simulink model "REAL_THREE_TANK"  (R2025b)
settings: Solver=ode15s  StartTime=0.0  StopTime=1500  RelTol=1e-3
InitFcn:
  | run("index.m")
StopFcn:
  | data_name = "realtime_data";
  | save_name = format_file_name(data_name,true);
  | 
  | % Save output data
  | save(save_name,"out")
values from neighbouring files (symbols this model uses):
  adaptParam = 0.15    [index.m]
  hiddenStates = 0    [index.m]
  model_const = struct()    [index.m]
undefined symbols (not defined in the file or in its folder): CR, LF, sigbuilder_block
libraries: instrumentseriallib x3, simulink x1
(part 1 of 2)
settings Model: Creator=HP  LastModifiedBy=USER PC
settings RTWCC: GPUComputeCapability=3.5
settings GRTTargetCC: ArrayLayout=Row-major

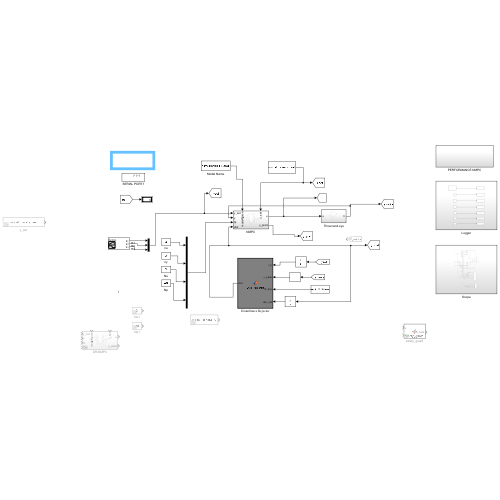
[thumbnail: Simulink's stored preview of the top-level diagram]
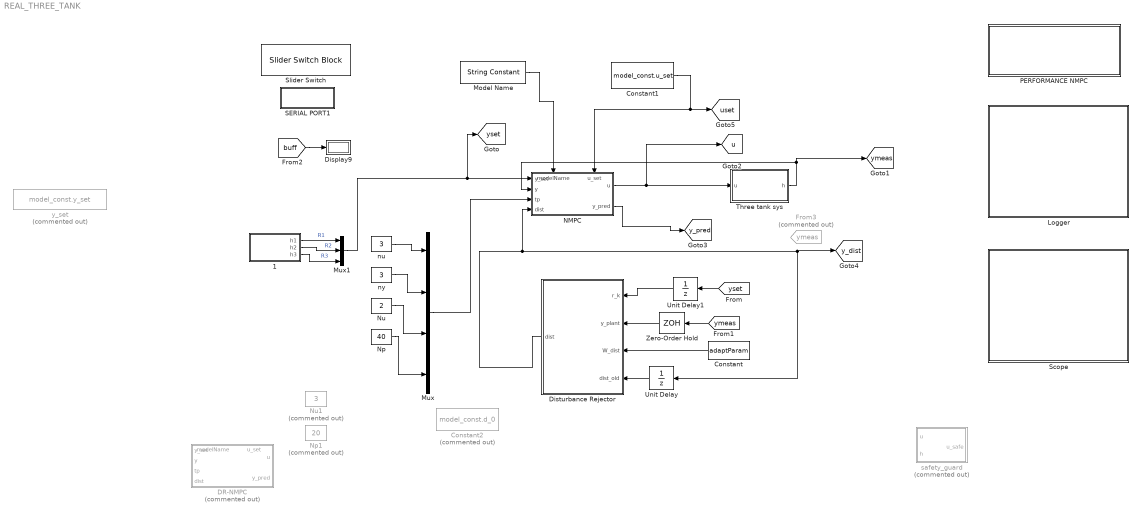
== system REAL_THREE_TANK ==
  " 1" : Subsystem  Tag=STV Subsys  LoadFcn=sigbuilder_block('load');  StartFcn=sigbuilder_block('start');  StopFcn=sigbuilder_block('stop');  ClipboardFcn=sigbuilder_block('clipboard');  mask(Sigbuilder block){tuvar=[0:10]}
      mask help: Simulink:masks:SigbuilderBlock_MD
      mask init:
      | if ~strcmp(get_param(bdroot(gcbh),'SimulationStatus'),'stopped') tuvar = sigbuilder_block('maskInit'); end
      settings: CopyFcn=sigbuilder_block('copy');  DeleteFcn=sigbuilder_block('delete');  ModelCloseFcn=sigbuilder_block('modelClose');  PreSaveFcn=sigbuilder_block('preSave');  PauseFcn=sigbuilder_block('pause');  ContinueFcn=sigbuilder_block('continue');  NameChangeFcn=sigbuilder_block('namechange');  OpenFcn=sigbuilder_block('open',[316.5 171.75 805.5 485.25 ]);  CloseFcn=sigbuilder_block('close');
      mask Display: plot(0, 0, 100, 100,[2, 2, 32, 32, 2], [68, 8, 8, 68, 68],[32, 2], [38, 38], [32, 19, 2],[53, 60, 44], [32, 17, 17, 2],[16, 16, 31, 31]);txt = getActiveGroup(gcbh);text(2, 100, txt,'verticalAlignment', 'top');
  Constant : Constant  Value=adaptParam
  Constant1 : Constant  Value=model_const.u_set  SampleTime=model_const.ts
  Constant2 : Constant  Commented=on  Value=model_const.d_0  SampleTime=model_const.ts
  DR-NMPC : Subsystem  Commented=on
      settings: PortSchema="{\"entries\":[{\"content\":{\"sides\":[{\"content\":{\"connectorIds\":[\"In1\",\"In2\",\"In3\",\"In4\"]},\"type\":\"ConnectorPlacement.EquallySpacedRectSide\",\"uuid\":\"b907109f-bf70-45ef-b014-879f3ccfb12e\"},{\"content\":{\"connectorIds\":[\"Out1\",\"Out2\"],\"side\":\"RIGHT\"},\"type\":\"ConnectorPlacement.EquallySpacedRectSide\",\"uuid\":\"26d01547-fbc3-4b4e-b6e6-c22ae9e5b6d6\"},{\"content\":{\"connectorIds\":[\"In5\",\"In6\"],\"side\":\"TOP\"},\"type\":\"ConnectorPlacement.EquallySpacedRectSide\",\"uuid\":\"f1d5a2c8-1fb2-4706-a136-ec661fe312a9\"}]},\"type\":\"ConnectorPlacement.EquallySpacedConnector\",\"uuid\":\"8e79e654-12d3-4871-a9fc-130c68b7f74a\"}],\"packageUris\":[\"http://schema.mathworks.com/mf0/Connector/R2020b\"],\"version\":\"1.0\"}"
  Display9 : Display
  Disturbance Rejector : MATLAB Function  TreatAsAtomicUnit=on  SystemSampleTime=10
  From3 : From  Commented=on  GotoTag=ymeas  TagVisibility=global
  Logger : Subsystem
  Model Name : StringConstant  String=networkModelName
  Mux : Mux
  Mux1 : Mux  Inputs=3
  NMPC : Subsystem
      settings: PortSchema="{\"entries\":[{\"content\":{\"sides\":[{\"content\":{\"connectorIds\":[\"In1\",\"In2\",\"In3\",\"In4\"]},\"type\":\"ConnectorPlacement.EquallySpacedRectSide\",\"uuid\":\"b907109f-bf70-45ef-b014-879f3ccfb12e\"},{\"content\":{\"connectorIds\":[\"Out1\",\"Out2\"],\"side\":\"RIGHT\"},\"type\":\"ConnectorPlacement.EquallySpacedRectSide\",\"uuid\":\"26d01547-fbc3-4b4e-b6e6-c22ae9e5b6d6\"},{\"content\":{\"connectorIds\":[\"In5\",\"In6\"],\"side\":\"TOP\"},\"type\":\"ConnectorPlacement.EquallySpacedRectSide\",\"uuid\":\"f1d5a2c8-1fb2-4706-a136-ec661fe312a9\"}]},\"type\":\"ConnectorPlacement.EquallySpacedConnector\",\"uuid\":\"8e79e654-12d3-4871-a9fc-130c68b7f74a\"}],\"packageUris\":[\"http://schema.mathworks.com/mf0/Connector/R2020b\"],\"version\":\"1.0\"}"
  Np : Constant  Value=40
  Np1 : Constant  Commented=on  Value=20
  Nu : Constant  Value=2
  Nu1 : Constant  Commented=on  Value=3
  PERFORMANCE NMPC : Subsystem
  SERIAL PORT1 : Subsystem
      mask Display: image('rs232.png');
  Scope : Subsystem
  Slider Switch : SliderSwitchBlock  LabelPosition=Hide
  Three tank sys : Subsystem
  Unit Delay : UnitDelay  InitialCondition=[0;0;0]  SampleTime=model_const.ts  HasFrameUpgradeWarning=on
  Unit Delay1 : UnitDelay  InitialCondition=[100; 0.4; 0.2]  SampleTime=model_const.ts  HasFrameUpgradeWarning=on
  Zero-Order Hold : ZeroOrderHold  SampleTime=model_const.ts
  nu : Constant  Value=3
  ny : Constant  Value=3
  safety_guard : MATLAB Function  Commented=on  TreatAsAtomicUnit=on
  y_set : Constant  Commented=on  Value=model_const.y_set  SampleTime=model_const.ts  LockScale=on
  tag scope: u=global, uset=global, y_dist=global, y_pred=global, ymeas=global, yset=global
  wires:
  Nu/1 -> Mux/3
  Constant/1 -> Disturbance Rejector/3(W_dist)
  Unit Delay/1 -> Disturbance Rejector/4(dist_old)
  Mux/1 -> NMPC/3(tp)
  Np/1 -> Mux/4
  [ymeas] -> Zero-Order Hold/1
  Model Name/1 -> NMPC/5(modelName)
  nu/1 -> Mux/1
  ny/1 -> Mux/2
  Constant1/1 -> NMPC/6(u_set), [uset]
  Disturbance Rejector/1(dist) -> NMPC/4(dist), [y_dist], Unit Delay/1
  [yset] -> Unit Delay1/1
  Three tank sys/1(h) -> NMPC/2(y), [ymeas]
  [buff] -> Display9/1
  " 1"/3(h3) -> Mux1/3  "R3"
  " 1"/2(h2) -> Mux1/2  "R2"
  " 1"/1(h1) -> Mux1/1  "R1"
  NMPC/2(y_pred) -> [y_pred]
  NMPC/1(u) -> Three tank sys/1(u), [u]
  Mux1/1 -> [yset], NMPC/1(y_set)
  Zero-Order Hold/1 -> Disturbance Rejector/2(y_plant)
  Unit Delay1/1 -> Disturbance Rejector/1(r_k)

== system REAL_THREE_TANK/ 1 ==
  Demux : Demux  Tag=STV Demux  Outputs=3
      settings: DisplayOption=none
  FromWs : FromWorkspace  Tag=STV FromWs  VariableName=tuvar  SampleTime=1
      SigBuilderData=|
      | common.afterFinalStr = 'Extrapolate'
      | common.sampleTime = '1'
      | dataSet.timeRange = [0 1500]
      | dataSet.name = 'Servo'
      | sbobj.Groups.Name = 'Servo'
      | sbobj.Groups.Signals(1).Name = 'h1'
      | sbobj.Groups.Signals(1).XData = [0 400 400 1500]
      | sbobj.Groups.Signals(1).YData = [14.29 14.29 20 20]
      | sbobj.Groups.Signals(2).Name = 'h2'
      | sbobj.Groups.Signals(2).XData = [0 800 800 1500]
      | sbobj.Groups.Signals(2).YData = [13.51 13.51 20 20]
      | sbobj.Groups.Signals(3).Name = 'h3'
      | sbobj.Groups.Signals(3).XData = [0 1200 1200 1500]
      | sbobj.Groups.Signals(3).YData = [16.06 16.06 20 20]
      | sbobj.Groups.TimeRange = [0 1500]
  h1 : Outport  Tag=STV Outport  VectorParamsAs1DForOutWhenUnconnected=off
  h2 : Outport  Tag=STV Outport  Port=2  VectorParamsAs1DForOutWhenUnconnected=off
  h3 : Outport  Tag=STV Outport  Port=3  VectorParamsAs1DForOutWhenUnconnected=off
  wires:
  FromWs/1 -> Demux/1
  Demux/1 -> h1/1
  Demux/2 -> h2/1
  Demux/3 -> h3/1

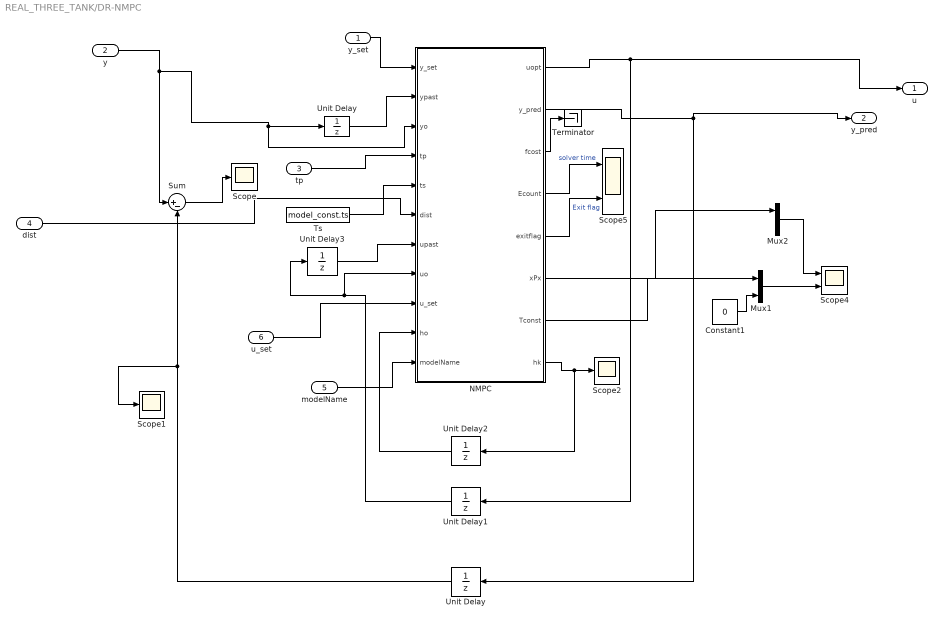
== system REAL_THREE_TANK/DR-NMPC ==
  y_set : Inport
  y : Inport  Port=2
  tp : Inport  Port=3
  dist : Inport  Port=4
  modelName : Inport  Port=5
  u_set : Inport  Port=6
  "  Unit Delay  " : UnitDelay  InitialCondition=model_const.y_0  SampleTime=model_const.ts  HasFrameUpgradeWarning=on
  " Unit Delay " : UnitDelay  InitialCondition=model_const.y_set  SampleTime=model_const.ts  HasFrameUpgradeWarning=on
  Constant1 : Constant  Value=0
  Mux1 : Mux  Inputs=2
  Mux2 : Mux  Inputs=2
  "NMPC " : MATLAB Function  TreatAsAtomicUnit=on  SystemSampleTime=model_const.ts
  Scope : Scope
      settings: ActiveDisplayYMinimum=-0.81983  ActiveDisplayYMaximum=1.85991
  Scope1 : Scope
      settings: ActiveDisplayYMinimum=2.45433  ActiveDisplayYMaximum=11.20291
  Scope2 : Scope
      settings: ActiveDisplayYMinimum=-0.0970614142715931  ActiveDisplayYMaximum=0.12913854792714119
  Scope4 : Scope  NumInputPorts=2
      settings: ActiveDisplayYMinimum=-0.25  ActiveDisplayYMaximum=2.25  DataLoggingVariableName=ScopeData2
  Scope5 : Scope  NumInputPorts=2
      settings: ShowGrid=off  ActiveDisplayYMinimum=-2.5  ActiveDisplayYMaximum=2.5  DataLoggingVariableName=ScopeData3
  Sum : Sum  Inputs=|+-
  "Terminator " : Terminator
  Ts : Constant  Value=model_const.ts
  Unit Delay1 : UnitDelay  InitialCondition=model_const.u_0  SampleTime=model_const.ts  HasFrameUpgradeWarning=on
  Unit Delay2 : UnitDelay  InitialCondition=hiddenStates  SampleTime=model_const.ts  HasFrameUpgradeWarning=on
  Unit Delay3 : UnitDelay  InitialCondition=model_const.u_0  SampleTime=model_const.ts  HasFrameUpgradeWarning=on
  u : Outport  VectorParamsAs1DForOutWhenUnconnected=off
  y_pred : Outport  Port=2  VectorParamsAs1DForOutWhenUnconnected=off
  wires:
  y_set/1 -> "NMPC "/1(y_set)
  tp/1 -> "NMPC "/4(tp)
  Ts/1 -> "NMPC "/5(ts)
  "NMPC "/3(fcost) -> "Terminator "/1
  y/1 -> Sum/1, "NMPC "/3(yo), " Unit Delay "/1
  "  Unit Delay  "/1 -> Scope1/1, Sum/2
  Sum/1 -> Scope/1
  dist/1 -> "NMPC "/6(dist)
  Constant1/1 -> Mux1/2
  Mux2/1 -> Scope4/1
  Mux1/1 -> Scope4/2
  "NMPC "/7(Tconst) -> Mux1/1
  "NMPC "/6(xPx) -> Mux2/1
  "NMPC "/4(Ecount) -> Scope5/1  "solver time"
  "NMPC "/5(exitflag) -> Scope5/2  "Exit flag"
  "NMPC "/8(hk) -> Unit Delay2/1, Scope2/1
  Unit Delay2/1 -> "NMPC "/10(ho)
  modelName/1 -> "NMPC "/11(modelName)
  "NMPC "/1(uopt) -> Unit Delay1/1, u/1
  Unit Delay1/1 -> Unit Delay3/1, "NMPC "/8(uo)
  " Unit Delay "/1 -> "NMPC "/2(ypast)
  Unit Delay3/1 -> "NMPC "/7(upast)
  u_set/1 -> "NMPC "/9(u_set)
  "NMPC "/2(y_pred) -> y_pred/1, "  Unit Delay  "/1

== system REAL_THREE_TANK/Logger ==
  String Constant : StringConstant  String=description
  To Workspace : ToWorkspace  VariableName=input  SaveFormat=Structure With Time  SampleTime=3
      settings: Decimation=2
  To Workspace1 : ToWorkspace  VariableName=desc  SaveFormat=Structure With Time  SampleTime=3
      settings: Decimation=2
  To Workspace2 : ToWorkspace  VariableName=input_set  SaveFormat=Structure With Time  SampleTime=3
      settings: Decimation=2
  To Workspace3 : ToWorkspace  VariableName=out_dist  SaveFormat=Structure With Time  SampleTime=3
      settings: Decimation=2
  To Workspace4 : ToWorkspace  VariableName=out_pred  SaveFormat=Structure With Time  SampleTime=3
      settings: Decimation=2
  To Workspace5 : ToWorkspace  VariableName=out_meas  SaveFormat=Structure With Time  SampleTime=3
      settings: Decimation=2
  To Workspace6 : ToWorkspace  VariableName=out_set  SaveFormat=Structure With Time  SampleTime=3
      settings: Decimation=2
  wires:
  [u] -> To Workspace/1
  [yset] -> To Workspace6/1
  [ymeas] -> To Workspace5/1
  [y_pred] -> To Workspace4/1
  [y_dist] -> To Workspace3/1
  [uset] -> To Workspace2/1
  String Constant/1 -> To Workspace1/1

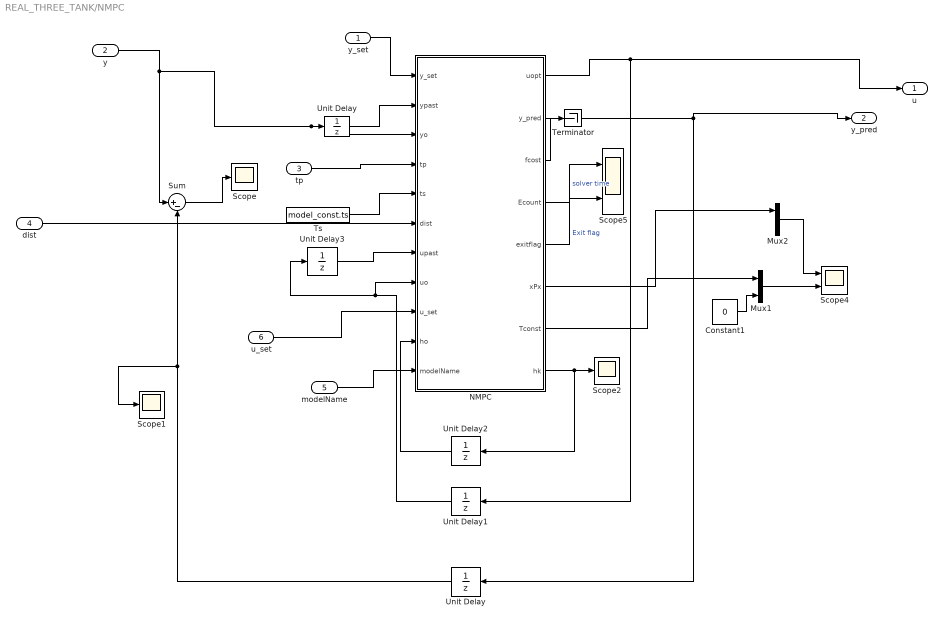
== system REAL_THREE_TANK/NMPC ==
  y_set : Inport
  y : Inport  Port=2
  tp : Inport  Port=3
  dist : Inport  Port=4
  modelName : Inport  Port=5
  u_set : Inport  Port=6
  "  Unit Delay  " : UnitDelay  InitialCondition=model_const.y_0  SampleTime=model_const.ts  HasFrameUpgradeWarning=on
  " Unit Delay " : UnitDelay  InitialCondition=[0 0 0]  SampleTime=model_const.ts  HasFrameUpgradeWarning=on
  Constant1 : Constant  Value=0
  Mux1 : Mux  Inputs=2
  Mux2 : Mux  Inputs=2
  "NMPC " : MATLAB Function  TreatAsAtomicUnit=on  SystemSampleTime=model_const.ts
  Scope : Scope
      settings: ActiveDisplayYMinimum=-0.81983  ActiveDisplayYMaximum=1.85991
  Scope1 : Scope
      settings: ActiveDisplayYMinimum=2.45433  ActiveDisplayYMaximum=11.20291
  Scope2 : Scope
      settings: ActiveDisplayYMinimum=-0.0970614142715931  ActiveDisplayYMaximum=0.12913854792714119
  Scope4 : Scope  NumInputPorts=2
      settings: ActiveDisplayYMinimum=-0.25  ActiveDisplayYMaximum=2.25  DataLoggingVariableName=ScopeData2
  Scope5 : Scope  NumInputPorts=2
      settings: ShowGrid=off  ActiveDisplayYMinimum=-2.5  ActiveDisplayYMaximum=2.5  DataLoggingVariableName=ScopeData3
  Sum : Sum  Inputs=|+-
  "Terminator " : Terminator
  Ts : Constant  Value=model_const.ts
  Unit Delay1 : UnitDelay  InitialCondition=model_const.u_0  SampleTime=model_const.ts  HasFrameUpgradeWarning=on
  Unit Delay2 : UnitDelay  InitialCondition=hiddenStates  SampleTime=model_const.ts  HasFrameUpgradeWarning=on
  Unit Delay3 : UnitDelay  InitialCondition=model_const.u_0  SampleTime=model_const.ts  HasFrameUpgradeWarning=on
  u : Outport  VectorParamsAs1DForOutWhenUnconnected=off
  y_pred : Outport  Port=2  VectorParamsAs1DForOutWhenUnconnected=off
  wires:
  y_set/1 -> "NMPC "/1(y_set)
  tp/1 -> "NMPC "/4(tp)
  Ts/1 -> "NMPC "/5(ts)
  "NMPC "/3(fcost) -> "Terminator "/1
  y/1 -> Sum/1, "NMPC "/3(yo), " Unit Delay "/1
  "  Unit Delay  "/1 -> Scope1/1, Sum/2
  Sum/1 -> Scope/1
  dist/1 -> "NMPC "/6(dist)
  Constant1/1 -> Mux1/2
  Mux2/1 -> Scope4/1
  Mux1/1 -> Scope4/2
  "NMPC "/7(Tconst) -> Mux1/1
  "NMPC "/6(xPx) -> Mux2/1
  "NMPC "/4(Ecount) -> Scope5/1  "solver time"
  "NMPC "/5(exitflag) -> Scope5/2  "Exit flag"
  "NMPC "/8(hk) -> Unit Delay2/1, Scope2/1
  Unit Delay2/1 -> "NMPC "/10(ho)
  modelName/1 -> "NMPC "/11(modelName)
  "NMPC "/1(uopt) -> Unit Delay1/1, u/1
  Unit Delay1/1 -> Unit Delay3/1, "NMPC "/8(uo)
  " Unit Delay "/1 -> "NMPC "/2(ypast)
  Unit Delay3/1 -> "NMPC "/7(upast)
  u_set/1 -> "NMPC "/9(u_set)
  "NMPC "/2(y_pred) -> y_pred/1, "  Unit Delay  "/1

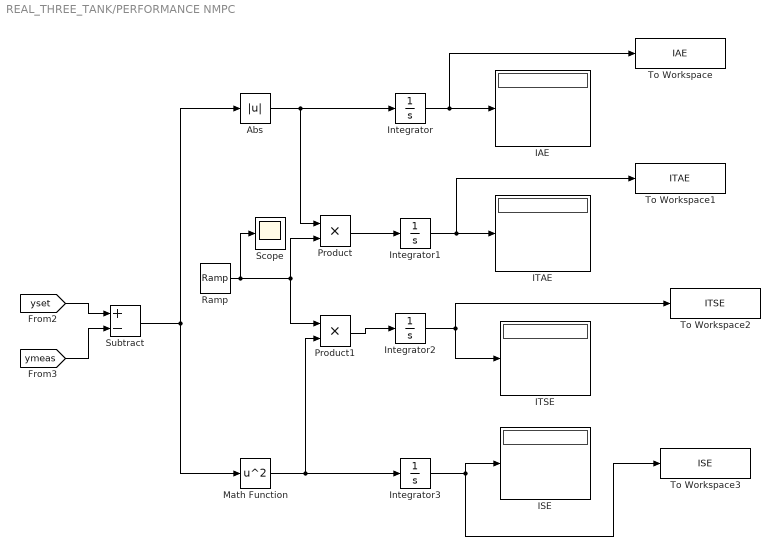
== system REAL_THREE_TANK/PERFORMANCE NMPC ==
  Abs : Abs  SaturateOnIntegerOverflow=off
  IAE : Display
  ISE : Display
  ITAE : Display
  ITSE : Display
  Integrator{,1..3} (4 alike) : Integrator
  Math Function : Math  Operator=square  SignedPower=on
  Product : Product  RndMeth=Zero
  Product1 : Product  RndMeth=Zero
  Ramp : simulink/Sources/Ramp  slope=1  start=0  InitialOutput=0
  Scope : Scope
      settings: DataLoggingSaveFormat=Array
  Subtract : Sum  Inputs=+-
  To Workspace : ToWorkspace  VariableName=IAE  SaveFormat=Structure With Time  SampleTime=3
      settings: Decimation=4
  To Workspace1 : ToWorkspace  VariableName=ITAE  SaveFormat=Structure With Time  SampleTime=3
      settings: Decimation=4
  To Workspace2 : ToWorkspace  VariableName=ITSE  SaveFormat=Structure With Time  SampleTime=3
      settings: Decimation=4
  To Workspace3 : ToWorkspace  VariableName=ISE  SaveFormat=Structure With Time  SampleTime=3
      settings: Decimation=4
  wires:
  Integrator1/1 -> To Workspace1/1, ITAE/1
  Integrator3/1 -> ISE/1, To Workspace3/1
  Product/1 -> Integrator1/1
  Product1/1 -> Integrator2/1
  Math Function/1 -> Product1/2, Integrator3/1
  Ramp/1 -> Scope/1, Product1/1, Product/2
  Integrator/1 -> To Workspace/1, IAE/1
  Abs/1 -> Product/1, Integrator/1
  Subtract/1 -> Abs/1, Math Function/1
  [yset] -> Subtract/1
  [ymeas] -> Subtract/2
  Integrator2/1 -> ITSE/1, To Workspace2/1

== system REAL_THREE_TANK/SERIAL PORT1 ==
  Display : Display
  Serial Configuration : instrumentseriallib/Serial Configuration  Priority=-200000  PortSel=COM10  Port=COM10  ComPort=COM10  BaudRate=115200  DataBits=8  Parity=none  StopBits=1  ByteOrder=little-endian  FlowControl=none  Timeout=3000  SimulateUsing=Interpreted execution  BlockInModel=on  aMode=1
  Serial Receive : instrumentseriallib/Serial Receive  Priority=1  PortSel=COM10  Port=COM10  ComPort=COM10  DataType=int8  SaveDataType=uint8  ToggleHeader=on  Header=[35 35]  ToggleDataSize=on  DataSize=[1 15]  ToggleTerminator=on  Terminator=CR/LF ('\r\n')  CustomTerminator=[]  InputFormat=Column major  EnableBlockingMode=off  ActionDataUnavailable=Output last received value  ActionWhenDataUnavailable=Output last received value  CustomValue=0  SampleTime=1  SimulateUsing=Interpreted execution  BlockInModel=on  aMode=1  LibraryInUse=instrumentlib
  Serial Send : instrumentseriallib/Serial Send  Priority=1  PortSel=COM10  Port=COM10  ComPort=COM10  Header=[]  Terminator=<none>  CustomTerminator=[]  EnableBlockingMode=on  SimulateUsing=Interpreted execution  BlockInModel=on  aMode=1
  To Workspace : ToWorkspace  VariableName=raw_read_sensor  SaveFormat=Structure With Time  SampleTime=-1
  To Workspace1 : ToWorkspace  VariableName=raw_read_status  SaveFormat=Structure With Time  SampleTime=-1
  tag scope: buff=global, rcv=global
  wires:
  Serial Receive/1 -> [rcv], To Workspace/1
  [send] -> Serial Send/1
  Serial Receive/2 -> To Workspace1/1, [buff], Display/1

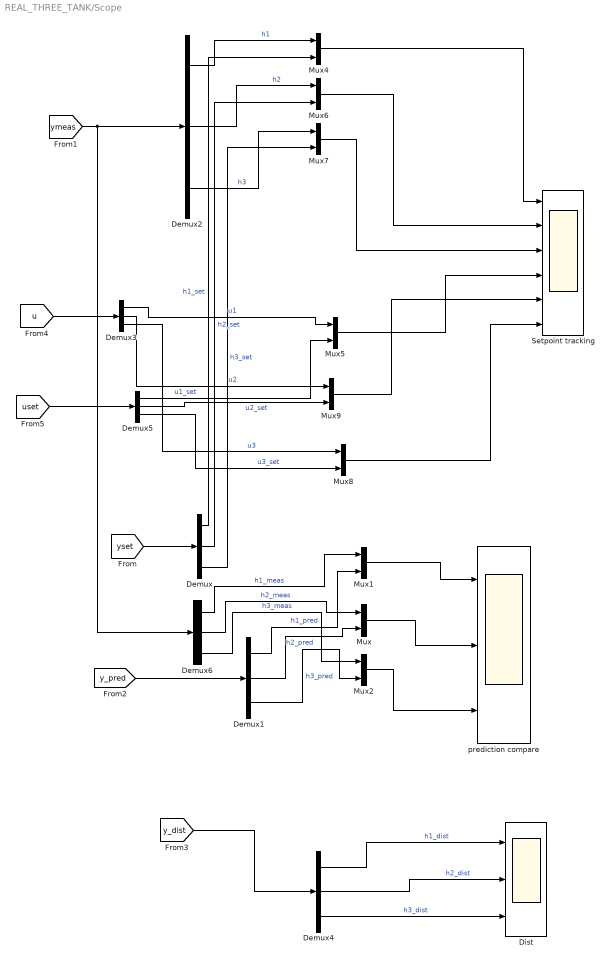
== system REAL_THREE_TANK/Scope ==
  Demux{,1..6} (7 alike) : Demux  Outputs=3
  Dist : Scope  NumInputPorts=3
      settings: ShowGrid=off  ActiveDisplayYMinimum=-17.700526540347088  ActiveDisplayYMaximum=9.30473886312379  DataLoggingVariableName=dist
  Mux{,1..2,4..9} (9 alike) : Mux  Inputs=2
  Setpoint tracking : Scope  NumInputPorts=6
      settings: SampleTime=model_const.ts  ActiveDisplayString=6  ShowGrid=off  ActiveDisplayYMinimum=0.015000000000000027  ActiveDisplayYMaximum=0.965  DataLoggingVariableName=servo
  prediction compare : Scope  NumInputPorts=3
      settings: SampleTime=model_const.ts  ShowGrid=off  ActiveDisplayYMinimum=-1.9430444010545433  ActiveDisplayYMaximum=17.487399609490893  DataLoggingVariableName=error
  wires:
  Demux/1 -> Mux4/2  "h1_set"
  Mux2/1 -> prediction compare/3
  Mux1/1 -> prediction compare/1
  [yset] -> Demux/1
  [y_pred] -> Demux1/1
  Demux1/1 -> Mux1/2  "h1_pred"
  Demux1/2 -> Mux/2  "h2_pred"
  Demux1/3 -> Mux2/2  "h3_pred"
  Demux/2 -> Mux6/2  "h2_set"
  Demux/3 -> Mux7/2  "h3_set"
  Mux/1 -> prediction compare/2
  [u] -> Demux3/1
  Demux3/1 -> Mux5/1  "u1"
  Demux3/2 -> Mux9/1  "u2"
  [ymeas] -> Demux6/1, Demux2/1
  Mux7/1 -> Setpoint tracking/3
  Mux6/1 -> Setpoint tracking/2
  Mux4/1 -> Setpoint tracking/1
  Demux2/1 -> Mux4/1  "h1"
  Demux2/2 -> Mux6/1  "h2"
  Demux2/3 -> Mux7/1  "h3"
  [y_dist] -> Demux4/1
  Demux4/1 -> Dist/1  "h1_dist"
  Demux4/2 -> Dist/2  "h2_dist"
  Demux4/3 -> Dist/3  "h3_dist"
  [uset] -> Demux5/1
  Demux5/1 -> Mux5/2  "u1_set"
  Demux5/2 -> Mux9/2  "u2_set"
  Mux5/1 -> Setpoint tracking/4
  Demux6/1 -> Mux1/1  "h1_meas"
  Demux6/2 -> Mux/1  "h2_meas"
  Demux6/3 -> Mux2/1  "h3_meas"
  Mux9/1 -> Setpoint tracking/5
  Mux8/1 -> Setpoint tracking/6
  Demux3/3 -> Mux8/1  "u3"
  Demux5/3 -> Mux8/2  "u3_set"

== system REAL_THREE_TANK/Three tank sys ==
  u : Inport
  " 1" : Subsystem  Tag=STV Subsys  LoadFcn=sigbuilder_block('load');  StartFcn=sigbuilder_block('start');  StopFcn=sigbuilder_block('stop');  ClipboardFcn=sigbuilder_block('clipboard');  mask(Sigbuilder block){tuvar=[0:10]}
      mask help: Simulink:masks:SigbuilderBlock_MD
      mask init:
      | if ~strcmp(get_param(bdroot(gcbh),'SimulationStatus'),'stopped') tuvar = sigbuilder_block('maskInit'); end
      settings: CopyFcn=sigbuilder_block('copy');  DeleteFcn=sigbuilder_block('delete');  ModelCloseFcn=sigbuilder_block('modelClose');  PreSaveFcn=sigbuilder_block('preSave');  PauseFcn=sigbuilder_block('pause');  ContinueFcn=sigbuilder_block('continue');  NameChangeFcn=sigbuilder_block('namechange');  OpenFcn=sigbuilder_block('open',[316.5 171.75 805.5 485.25 ]);  CloseFcn=sigbuilder_block('close');
      mask Display: plot(0, 0, 100, 100,[2, 2, 32, 32, 2], [68, 8, 8, 68, 68],[32, 2], [38, 38], [32, 19, 2],[53, 60, 44], [32, 17, 17, 2],[16, 16, 31, 31]);txt = getActiveGroup(gcbh);text(2, 100, txt,'verticalAlignment', 'top');
  Constant20 : Constant
  Demux : Demux  Outputs=3
  Mux : Mux  Inputs=3
  THREE_TANKS REALTIME_ PLANT : Subsystem
  c2 : Constant  Commented=on  Value=0.333
  "c3 " : Constant  Commented=on  Value=0.333
  h : Outport
  wires:
  Demux/2 -> THREE_TANKS REALTIME_ PLANT/2(U2)
  u/1 -> Demux/1
  Demux/3 -> THREE_TANKS REALTIME_ PLANT/3(U3)
  Demux/1 -> THREE_TANKS REALTIME_ PLANT/1(U1)
  THREE_TANKS REALTIME_ PLANT/1(H1) -> Mux/1  "h1"
  THREE_TANKS REALTIME_ PLANT/2(H2) -> Mux/2  "h2"
  THREE_TANKS REALTIME_ PLANT/3(H3) -> Mux/3  "h3"
  Constant20/1 -> THREE_TANKS REALTIME_ PLANT/6(In1)
  Mux/1 -> h/1
  " 1"/1(C2) -> THREE_TANKS REALTIME_ PLANT/4(D1)
  " 1"/2(C3) -> THREE_TANKS REALTIME_ PLANT/5(D2)

== system REAL_THREE_TANK/Three tank sys/ 1 ==
  Demux : Demux  Tag=STV Demux  Outputs=2
      settings: DisplayOption=none
  FromWs : FromWorkspace  Tag=STV FromWs  VariableName=tuvar  SampleTime=1
      SigBuilderData=|
      | common.afterFinalStr = 'Extrapolate'
      | common.sampleTime = '1'
      | dataSet.timeRange = [0 2500]
      | dataSet.name = 'Regulatory'
      | sbobj.Groups.Name = 'Regulatory'
      | sbobj.Groups.Signals(1).Name = 'C2'
      | sbobj.Groups.Signals(1).XData = [0 505 505 1500 1500 2500]
      | sbobj.Groups.Signals(1).YData = [0.333 0.333 0 -0.006 0.333 0.333]
      | sbobj.Groups.Signals(2).Name = 'C3'
      | sbobj.Groups.Signals(2).XData = [0 1005 1005 2005 2005 2500]
      | sbobj.Groups.Signals(2).YData = [0.333 0.333 0.25 0.25 0.33 0.33]
      | sbobj.Groups.TimeRange = [0 2500]
  C2 : Outport  Tag=STV Outport  VectorParamsAs1DForOutWhenUnconnected=off
  C3 : Outport  Tag=STV Outport  Port=2  VectorParamsAs1DForOutWhenUnconnected=off
  wires:
  FromWs/1 -> Demux/1
  Demux/1 -> C2/1
  Demux/2 -> C3/1

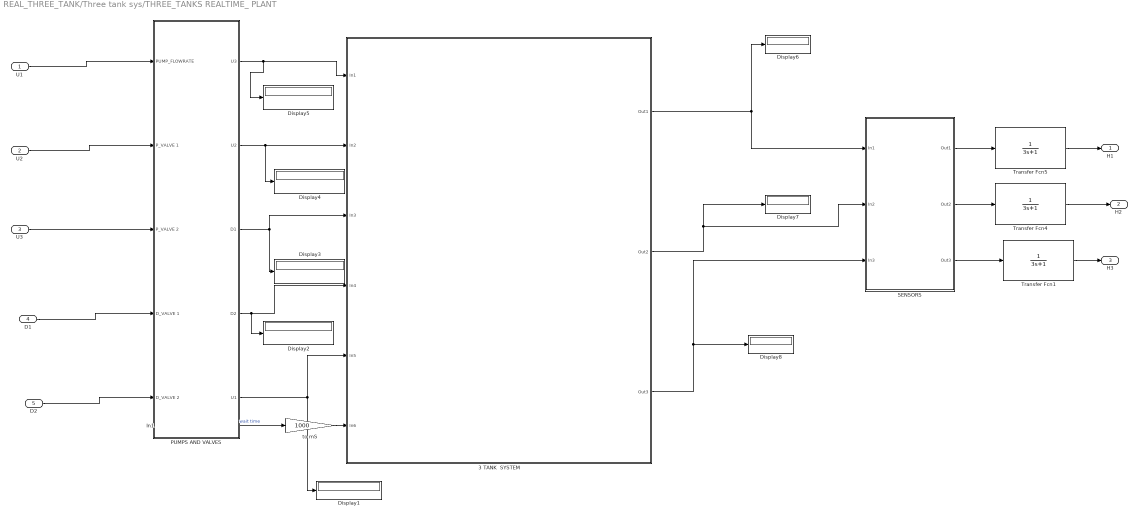
== system REAL_THREE_TANK/Three tank sys/THREE_TANKS REALTIME_ PLANT ==
  U1 : Inport
  U2 : Inport  Port=2
  U3 : Inport  Port=3
  D1 : Inport  Port=4
  D2 : Inport  Port=5
  In1 : Inport  Port=6
  "3 TANK  SYSTEM " : Subsystem  mask{Parameter1=}
      mask prompts: Parameter1 "This block represents the 3 Tank system"
      mask help: 3 TANK SYSTEM.
      mask Help: The inputs are the signal inputs to the 2 proportional values and the 2  , 4-position values. the out puts are raw values from the 3  water level sensors.
      mask Display: image('instrumentation.png');
  Display{1..8} (8 alike) : Display
  PUMPS AND VALVES : Subsystem
  SENSORS : Subsystem
  Transfer Fcn1 : TransferFcn  Denominator=[3 1]
  Transfer Fcn4 : TransferFcn  Denominator=[3 1]
  Transfer Fcn5 : TransferFcn  Denominator=[3 1]
  to mS : Gain  Gain=1000
  H1 : Outport  VectorParamsAs1DForOutWhenUnconnected=off
  H2 : Outport  Port=2  VectorParamsAs1DForOutWhenUnconnected=off
  H3 : Outport  Port=3  VectorParamsAs1DForOutWhenUnconnected=off
  wires:
  "3 TANK  SYSTEM "/3(Out3) -> SENSORS/3(In3), Display8/1
  PUMPS AND VALVES/4(D2) -> "3 TANK  SYSTEM "/4(In4), Display2/1
  PUMPS AND VALVES/2(U2) -> Display4/1, "3 TANK  SYSTEM "/2(In2)
  PUMPS AND VALVES/3(D1) -> Display3/1, "3 TANK  SYSTEM "/3(In3)
  SENSORS/2(Out2) -> Transfer Fcn4/1
  "3 TANK  SYSTEM "/2(Out2) -> Display7/1, SENSORS/2(In2)
  "3 TANK  SYSTEM "/1(Out1) -> Display6/1, SENSORS/1(In1)
  SENSORS/3(Out3) -> Transfer Fcn1/1
  SENSORS/1(Out1) -> Transfer Fcn5/1
  U2/1 -> PUMPS AND VALVES/2(P_VALVE 1)
  U3/1 -> PUMPS AND VALVES/3(P_VALVE 2)
  D1/1 -> PUMPS AND VALVES/4(D_VALVE 1)
  D2/1 -> PUMPS AND VALVES/5(D_VALVE 2)
  In1/1 -> to mS/1  "wait time"
  to mS/1 -> "3 TANK  SYSTEM "/6(In6)
  U1/1 -> PUMPS AND VALVES/1(PUMP_FLOWRATE)
  Transfer Fcn4/1 -> H2/1
  Transfer Fcn1/1 -> H3/1
  Transfer Fcn5/1 -> H1/1
  PUMPS AND VALVES/1(U3) -> "3 TANK  SYSTEM "/1(In1), Display5/1
  PUMPS AND VALVES/5(U1) -> "3 TANK  SYSTEM "/5(In5), Display1/1

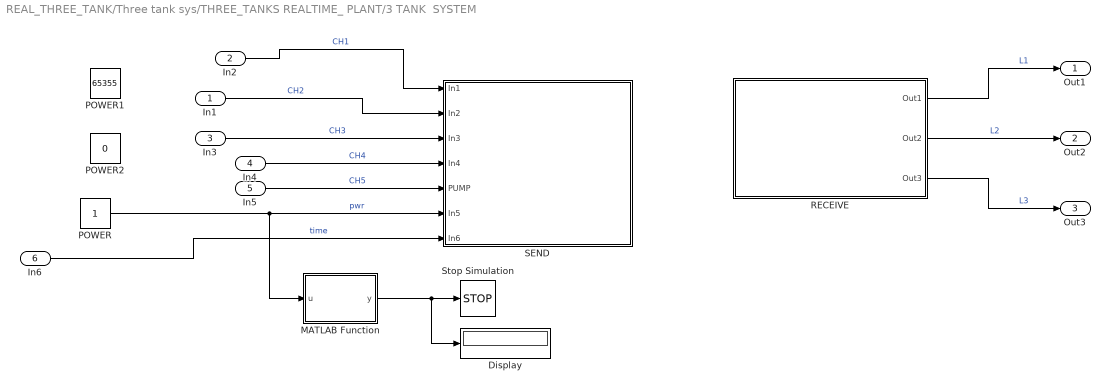
== system REAL_THREE_TANK/Three tank sys/THREE_TANKS REALTIME_ PLANT/3 TANK  SYSTEM  ==
  In1 : Inport
  In2 : Inport  Port=2
  In3 : Inport  Port=3
  In4 : Inport  Port=4
  In5 : Inport  Port=5
  In6 : Inport  Port=6
  Display : Display
  MATLAB Function : MATLAB Function  TreatAsAtomicUnit=on
  POWER : Constant
  POWER1 : Constant  Value=65355
  POWER2 : Constant  Value=0
  RECEIVE : Subsystem
      mask Display:
      | image('rs232.png');
      | text(0,10,'SERIAL PORT');
  SEND : Subsystem
      mask help: Serial port
      mask Display:
      | image('rs232.png');
      | text(0,10, 'SERIAL PORT');
  Stop Simulation : Stop
  Out1 : Outport  VectorParamsAs1DForOutWhenUnconnected=off
  Out2 : Outport  Port=2  VectorParamsAs1DForOutWhenUnconnected=off
  Out3 : Outport  Port=3  VectorParamsAs1DForOutWhenUnconnected=off
  wires:
  In1/1 -> SEND/2(In2)  "CH2"
  RECEIVE/2(Out2) -> Out2/1  "L2"
  In4/1 -> SEND/4(In4)  "CH4"
  RECEIVE/3(Out3) -> Out3/1  "L3"
  RECEIVE/1(Out1) -> Out1/1  "L1"
  In2/1 -> SEND/1(In1)  "CH1"
  In5/1 -> SEND/5(PUMP)  "CH5"
  In3/1 -> SEND/3(In3)  "CH3"
  POWER/1 -> MATLAB Function/1(u), SEND/6(In5)  "pwr"
  MATLAB Function/1(y) -> Display/1, Stop Simulation/1
  In6/1 -> SEND/7(In6)  "time"

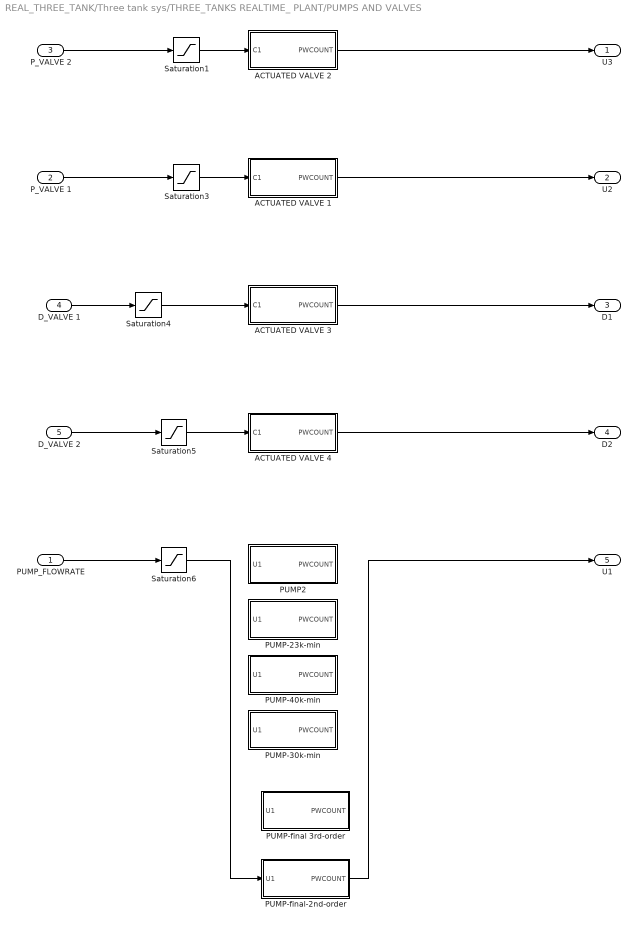
== system REAL_THREE_TANK/Three tank sys/THREE_TANKS REALTIME_ PLANT/PUMPS AND VALVES ==
  PUMP_FLOWRATE : Inport
  P_VALVE 1 : Inport  Port=2
  P_VALVE 2 : Inport  Port=3
  D_VALVE 1 : Inport  Port=4
  D_VALVE 2 : Inport  Port=5
  ACTUATED VALVE 1 : Subsystem
  ACTUATED VALVE 2 : Subsystem
  ACTUATED VALVE 3 : Subsystem
  ACTUATED VALVE 4 : Subsystem
  PUMP-23k-min : Subsystem
  PUMP-30k-min : Subsystem
  PUMP-40k-min : Subsystem
  PUMP-final 3rd-order : Subsystem
  PUMP-final-2nd-order : Subsystem
  PUMP2 : Subsystem
  Saturation{1,3..5} (4 alike) : Saturate  UpperLimit=1  LowerLimit=0
  Saturation6 : Saturate  UpperLimit=230  LowerLimit=0
  U3 : Outport  VectorParamsAs1DForOutWhenUnconnected=off
  U2 : Outport  Port=2  VectorParamsAs1DForOutWhenUnconnected=off
  D1 : Outport  Port=3  VectorParamsAs1DForOutWhenUnconnected=off
  D2 : Outport  Port=4  VectorParamsAs1DForOutWhenUnconnected=off
  U1 : Outport  Port=5  VectorParamsAs1DForOutWhenUnconnected=off
  wires:
  P_VALVE 2/1 -> Saturation1/1
  P_VALVE 1/1 -> Saturation3/1
  PUMP_FLOWRATE/1 -> Saturation6/1
  D_VALVE 1/1 -> Saturation4/1
  D_VALVE 2/1 -> Saturation5/1
  ACTUATED VALVE 2/1(PWCOUNT) -> U3/1
  ACTUATED VALVE 1/1(PWCOUNT) -> U2/1
  ACTUATED VALVE 3/1(PWCOUNT) -> D1/1
  ACTUATED VALVE 4/1(PWCOUNT) -> D2/1
  PUMP-final-2nd-order/1(PWCOUNT) -> U1/1
  Saturation6/1 -> PUMP-final-2nd-order/1(U1)
  Saturation5/1 -> ACTUATED VALVE 4/1(C1)
  Saturation4/1 -> ACTUATED VALVE 3/1(C1)
  Saturation3/1 -> ACTUATED VALVE 1/1(C1)
  Saturation1/1 -> ACTUATED VALVE 2/1(C1)

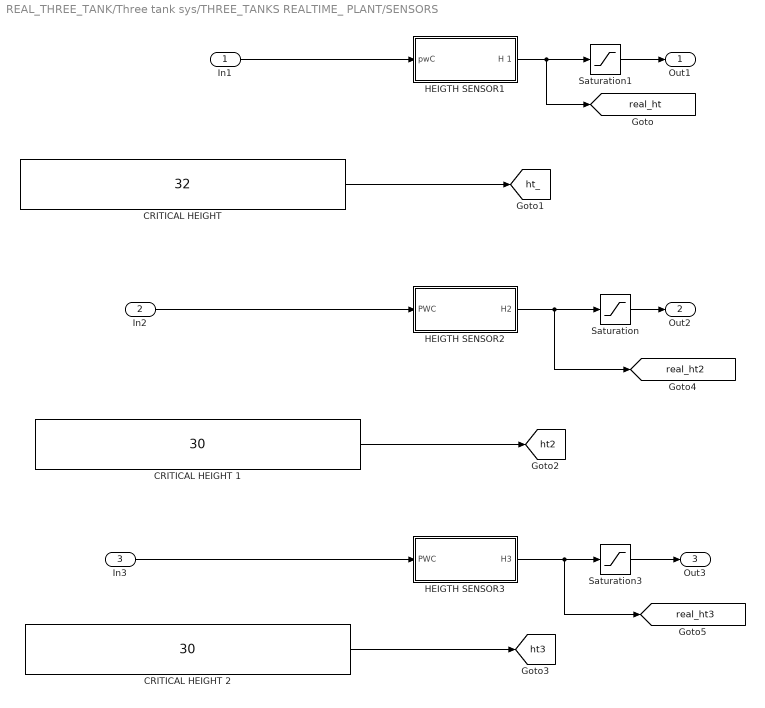
== system REAL_THREE_TANK/Three tank sys/THREE_TANKS REALTIME_ PLANT/SENSORS ==
  In1 : Inport
  In2 : Inport  Port=2
  In3 : Inport  Port=3
  "CRITICAL HEIGHT " : Constant  Value=32
  CRITICAL HEIGHT 1 : Constant  Value=30
  CRITICAL HEIGHT 2 : Constant  Value=30
  HEIGTH SENSOR1 : Subsystem
  HEIGTH SENSOR2 : Subsystem
  HEIGTH SENSOR3 : Subsystem
  Saturation : Saturate  UpperLimit=35  LowerLimit=0
  Saturation1 : Saturate  UpperLimit=35  LowerLimit=0
  Saturation3 : Saturate  UpperLimit=35  LowerLimit=0
  Out1 : Outport  VectorParamsAs1DForOutWhenUnconnected=off
  Out2 : Outport  Port=2  VectorParamsAs1DForOutWhenUnconnected=off
  Out3 : Outport  Port=3  VectorParamsAs1DForOutWhenUnconnected=off
  tag scope: ht2=global, ht3=global, ht_=global, real_ht2=global, real_ht3=global, real_ht=global
  wires:
  HEIGTH SENSOR2/1(H2) -> [real_ht2], Saturation/1
  HEIGTH SENSOR1/1(H 1) -> [real_ht], Saturation1/1
  HEIGTH SENSOR3/1(H3) -> [real_ht3], Saturation3/1
  In1/1 -> HEIGTH SENSOR1/1(pwC)
  In3/1 -> HEIGTH SENSOR3/1(PWC)
  In2/1 -> HEIGTH SENSOR2/1(PWC)
  "CRITICAL HEIGHT "/1 -> [ht_]
  Saturation/1 -> Out2/1
  Saturation1/1 -> Out1/1
  Saturation3/1 -> Out3/1
  CRITICAL HEIGHT 1/1 -> [ht2]
  CRITICAL HEIGHT 2/1 -> [ht3]

== system REAL_THREE_TANK/Three tank sys/THREE_TANKS REALTIME_ PLANT/3 TANK  SYSTEM /RECEIVE ==
  Demux2 : Demux  Outputs=15
  Display{,1..3} (4 alike) : Display
  Saturation1 : Saturate  UpperLimit=4098  LowerLimit=0
  Saturation2 : Saturate  UpperLimit=4098  LowerLimit=0
  Saturation3 : Saturate  UpperLimit=4098  LowerLimit=0
  Subsystem1 : Subsystem
  Subsystem2 : Subsystem
  Subsystem4 : Subsystem
  Out1 : Outport  VectorParamsAs1DForOutWhenUnconnected=off
  Out2 : Outport  Port=2  VectorParamsAs1DForOutWhenUnconnected=off
  Out3 : Outport  Port=3  VectorParamsAs1DForOutWhenUnconnected=off
  wires:
  [rcv] -> Demux2/1, Display/1
  Demux2/2 -> Subsystem1/1(In2)
  Demux2/3 -> Subsystem1/2(In3)
  Demux2/4 -> Subsystem1/3(In4)
  Demux2/5 -> Subsystem1/4(In5)
  Subsystem1/1(Out1) -> Saturation3/1
  Demux2/7 -> Subsystem2/1(In2)
  Demux2/8 -> Subsystem2/2(In3)
  Demux2/9 -> Subsystem2/3(In4)
  Demux2/10 -> Subsystem2/4(In5)
  Subsystem2/1(Out1) -> Saturation2/1
  Subsystem4/1(Out1) -> Saturation1/1
  Demux2/12 -> Subsystem4/1(In2)
  Demux2/13 -> Subsystem4/2(In3)
  Demux2/14 -> Subsystem4/3(In4)
  Demux2/15 -> Subsystem4/4(In5)
  Saturation1/1 -> Out3/1, Display3/1
  Saturation2/1 -> Out2/1, Display2/1
  Saturation3/1 -> Out1/1, Display1/1

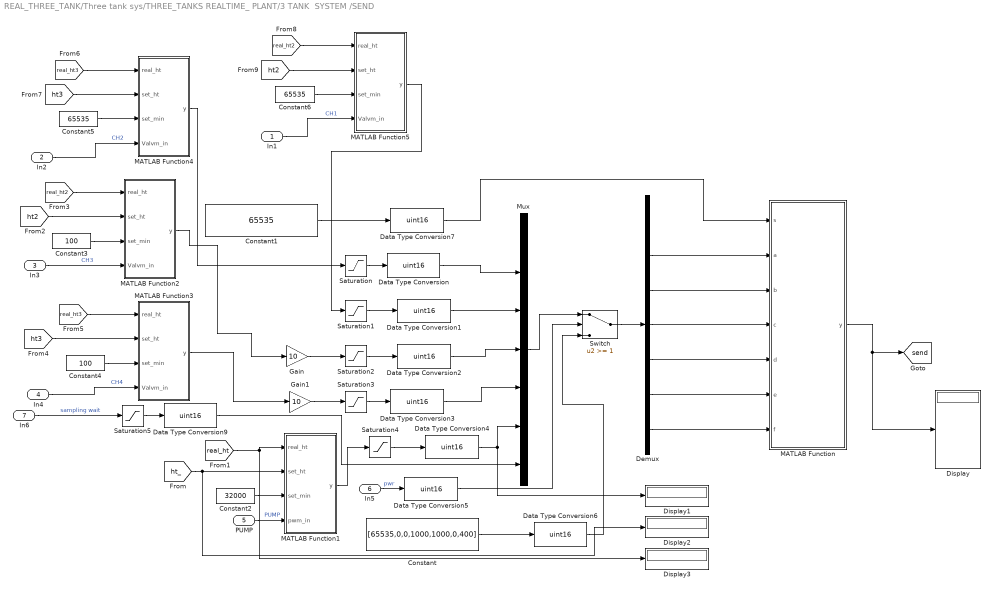
== system REAL_THREE_TANK/Three tank sys/THREE_TANKS REALTIME_ PLANT/3 TANK  SYSTEM /SEND ==
  In1 : Inport
  In2 : Inport  Port=2
  In3 : Inport  Port=3
  In4 : Inport  Port=4
  PUMP : Inport  Port=5
  In5 : Inport  Port=6
  In6 : Inport  Port=7
  Constant : Constant  Value=[65535,0,0,1000,1000,0,400]
  Constant1 : Constant  Value=65535
  Constant2 : Constant  Value=32000
  Constant3 : Constant  Value=100
  Constant4 : Constant  Value=100
  Constant5 : Constant  Value=65535
  Constant6 : Constant  Value=65535
  Data Type Conversion{,1..7,9} (9 alike) : DataTypeConversion  OutDataTypeStr=uint16  SaturateOnIntegerOverflow=off  RndMeth=Floor
  Demux : Demux  Outputs=7
  Display{,1..3} (4 alike) : Display
      settings: Format=decimal (Stored Integer)
  Gain : Gain  Gain=10
  Gain1 : Gain  Gain=10
  MATLAB Function : MATLAB Function  TreatAsAtomicUnit=on
  MATLAB Function1 : MATLAB Function  TreatAsAtomicUnit=on
  MATLAB Function2 : MATLAB Function  TreatAsAtomicUnit=on
  MATLAB Function3 : MATLAB Function  TreatAsAtomicUnit=on
  MATLAB Function4 : MATLAB Function  TreatAsAtomicUnit=on
  MATLAB Function5 : MATLAB Function  TreatAsAtomicUnit=on
  Mux : Mux  Inputs=7
  Saturation : Saturate  UpperLimit=65534  LowerLimit=0  LinearizeAsGain=off  ZeroCross=off
  Saturation1 : Saturate  UpperLimit=65534  LowerLimit=0  LinearizeAsGain=off  ZeroCross=off
  Saturation2 : Saturate  UpperLimit=1000  LowerLimit=0  LinearizeAsGain=off  ZeroCross=off
  Saturation3 : Saturate  UpperLimit=1000  LowerLimit=0  LinearizeAsGain=off  ZeroCross=off
  Saturation4 : Saturate  UpperLimit=65534  LowerLimit=0  LinearizeAsGain=off  ZeroCross=off
  Saturation5 : Saturate  UpperLimit=60000  LowerLimit=0  LinearizeAsGain=off  ZeroCross=off
  Switch : Switch  Threshold=1  SaturateOnIntegerOverflow=off  InputSameDT=off
  tag scope: send=global
  wires:
  In1/1 -> MATLAB Function5/4(Valvm_in)  "CH1"
  MATLAB Function/1(y) -> Display/1, [send]
  In2/1 -> MATLAB Function4/4(Valvm_in)  "CH2"
  In3/1 -> MATLAB Function2/4(Valvm_in)  "CH3"
  In4/1 -> MATLAB Function3/4(Valvm_in)  "CH4"
  In5/1 -> Data Type Conversion5/1  "pwr"
  Data Type Conversion5/1 -> Switch/2
  Data Type Conversion6/1 -> Switch/3
  Constant/1 -> Data Type Conversion6/1
  Demux/2 -> MATLAB Function/2(a)
  Demux/3 -> MATLAB Function/3(b)
  Demux/4 -> MATLAB Function/4(c)
  Demux/5 -> MATLAB Function/5(d)
  Demux/6 -> MATLAB Function/6(e)
  Data Type Conversion/1 -> Mux/2
  Data Type Conversion1/1 -> Mux/3
  Data Type Conversion2/1 -> Mux/4
  Data Type Conversion3/1 -> Mux/5
  Data Type Conversion4/1 -> Display1/1, Mux/6
  Switch/1 -> Demux/1
  Mux/1 -> Switch/1
  Data Type Conversion7/1 -> MATLAB Function/1(s)
  Constant1/1 -> Data Type Conversion7/1
  Saturation/1 -> Data Type Conversion/1
  Saturation1/1 -> Data Type Conversion1/1
  Saturation2/1 -> Data Type Conversion2/1
  Saturation3/1 -> Data Type Conversion3/1
  Saturation4/1 -> Data Type Conversion4/1
  Gain/1 -> Saturation2/1
  Gain1/1 -> Saturation3/1
  Constant2/1 -> MATLAB Function1/3(set_min)
  MATLAB Function1/1(y) -> Saturation4/1
  [ht_] -> Display2/1, MATLAB Function1/2(set_ht)
  [real_ht] -> Display3/1, MATLAB Function1/1(real_ht)
  PUMP/1 -> MATLAB Function1/4(pwm_in)  "PUMP"
  In6/1 -> Saturation5/1  "sampling wait"
  Saturation5/1 -> Data Type Conversion9/1
  Data Type Conversion9/1 -> Mux/7
  Demux/7 -> MATLAB Function/7(f)
  MATLAB Function2/1(y) -> Gain/1
  Constant3/1 -> MATLAB Function2/3(set_min)
  [ht2] -> MATLAB Function2/2(set_ht)
  [real_ht2] -> MATLAB Function2/1(real_ht)
  [real_ht3] -> MATLAB Function3/1(real_ht)
  [ht3] -> MATLAB Function3/2(set_ht)
  Constant4/1 -> MATLAB Function3/3(set_min)
  MATLAB Function3/1(y) -> Gain1/1
  [real_ht3] -> MATLAB Function4/1(real_ht)
  [ht3] -> MATLAB Function4/2(set_ht)
  Constant5/1 -> MATLAB Function4/3(set_min)
  [real_ht2] -> MATLAB Function5/1(real_ht)
  Constant6/1 -> MATLAB Function5/3(set_min)
  [ht2] -> MATLAB Function5/2(set_ht)
  MATLAB Function4/1(y) -> Saturation/1
  MATLAB Function5/1(y) -> Saturation1/1

== system REAL_THREE_TANK/Three tank sys/THREE_TANKS REALTIME_ PLANT/PUMPS AND VALVES/ACTUATED VALVE 1 ==
  C1 : Inport
  Add : Sum  Inputs=+++
  Constant : Constant  Value=52578
  Constant1 : Constant  Value=10759-3000
  Constant2 : Constant  Value=9000
  Constant3 : Constant  Value=10759
  Display : Display
  Gain1 : Gain  Gain=2343
  Math Function1 : Math  Operator=square  SignedPower=on
  Product : Product
  Saturation3 : Saturate  UpperLimit=65535  LowerLimit=10759
  Scope : Scope
      settings: DataLoggingVariableName=ScopeData2
  PWCOUNT : Outport  VectorParamsAs1DForOutWhenUnconnected=off
  wires:
  Constant2/1 -> Add/3
  Math Function1/1 -> Gain1/1
  C1/1 -> Math Function1/1, Product/1
  Add/1 -> Saturation3/1
  Constant/1 -> Product/2
  Product/1 -> Add/2
  Gain1/1 -> Add/1
  Saturation3/1 -> Display/1, Scope/1, PWCOUNT/1

== system REAL_THREE_TANK/Three tank sys/THREE_TANKS REALTIME_ PLANT/PUMPS AND VALVES/ACTUATED VALVE 2 ==
  note: p1 = 709.3 p2 = 54497 p3 = 12615
  C1 : Inport
  Add : Sum  Inputs=+++
  Constant : Constant  Value=54497
  Constant1 : Constant  Value=12615
  Constant2 : Constant  Value=52255
  Constant3 : Constant  Value=10771
  Constant4 : Constant  Value=40000
  Display : Display
  Gain1 : Gain  Gain=709.3
  Gain2 : Gain  Gain=2441.2
  Math Function1 : Math  Operator=square  SignedPower=on
  Product : Product
  Saturation3 : Saturate  UpperLimit=65535  LowerLimit=0
  Scope : Scope
      settings: DataLoggingVariableName=ScopeData3
  PWCOUNT : Outport  VectorParamsAs1DForOutWhenUnconnected=off
  wires:
  C1/1 -> Math Function1/1, Product/1
  Product/1 -> Add/2
  Add/1 -> Saturation3/1
  Constant/1 -> Product/2
  Math Function1/1 -> Gain1/1
  Gain1/1 -> Add/1
  Constant1/1 -> Add/3
  Saturation3/1 -> Display/1, Scope/1, PWCOUNT/1

== system REAL_THREE_TANK/Three tank sys/THREE_TANKS REALTIME_ PLANT/PUMPS AND VALVES/ACTUATED VALVE 3 ==
  C1 : Inport
  Constant1 : Constant  Value=100
  Display : Display
  Divide : Product  Inputs=**
  Scope : Scope
      settings: DataLoggingVariableName=ScopeData2
  PWCOUNT : Outport  VectorParamsAs1DForOutWhenUnconnected=off
  wires:
  Divide/1 -> Display/1, PWCOUNT/1, Scope/1
  C1/1 -> Divide/1
  Constant1/1 -> Divide/2

== system REAL_THREE_TANK/Three tank sys/THREE_TANKS REALTIME_ PLANT/PUMPS AND VALVES/ACTUATED VALVE 4 ==
  C1 : Inport
  Constant : Constant  Value=100
  Display : Display
  Product : Product
  Scope : Scope
      settings: DataLoggingVariableName=ScopeData2
  PWCOUNT : Outport  VectorParamsAs1DForOutWhenUnconnected=off
  wires:
  C1/1 -> Product/1
  Constant/1 -> Product/2
  Product/1 -> Scope/1, Display/1, PWCOUNT/1

== system REAL_THREE_TANK/Three tank sys/THREE_TANKS REALTIME_ PLANT/PUMPS AND VALVES/PUMP-23k-min ==
  note: p1 = 0.0047 p2 = -0.4981 p3 = 45.375 p4 = 37953
  U1 : Inport
  Add : Sum  Inputs=+++
  Constant : Constant  Value=10.897
  Constant1 : Constant  Value=22951
  Display : Display
  Gain1 : Gain  Gain=0.5085
  Math Function1 : Math  Operator=square  SignedPower=on
  Product : Product
  Saturation3 : Saturate  UpperLimit=55000  LowerLimit=23000
  Saturation6 : Saturate  UpperLimit=250  LowerLimit=0
  Scope : Scope
  PWCOUNT : Outport  VectorParamsAs1DForOutWhenUnconnected=off
  wires:
  Add/1 -> Saturation3/1
  U1/1 -> Saturation6/1
  Constant/1 -> Product/2
  Math Function1/1 -> Gain1/1
  Gain1/1 -> Add/1
  Product/1 -> Add/2
  Constant1/1 -> Add/3
  Saturation6/1 -> Math Function1/1, Product/1
  Saturation3/1 -> Display/1, Scope/1, PWCOUNT/1

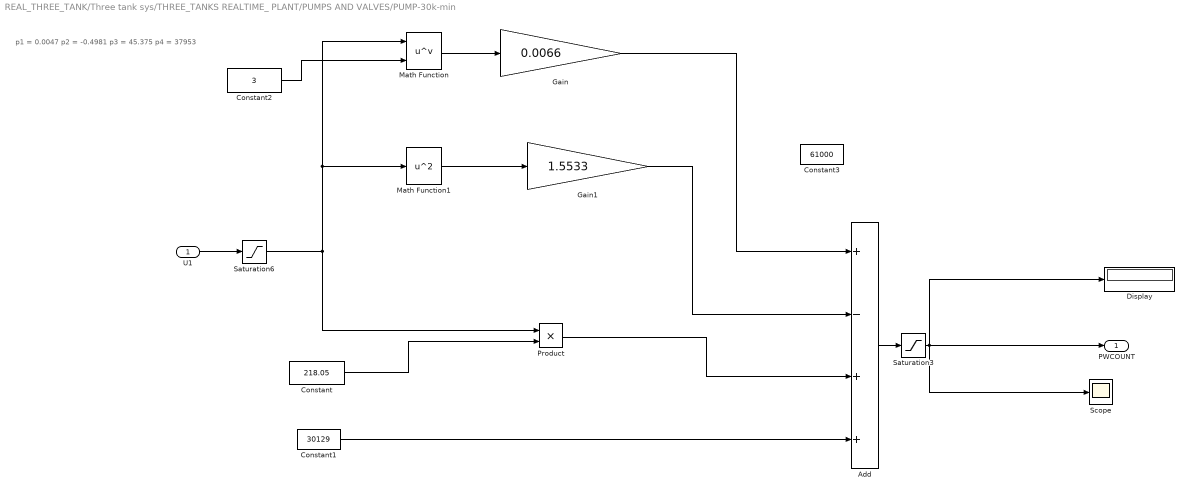
== system REAL_THREE_TANK/Three tank sys/THREE_TANKS REALTIME_ PLANT/PUMPS AND VALVES/PUMP-30k-min ==
  note: p1 = 0.0047 p2 = -0.4981 p3 = 45.375 p4 = 37953
  U1 : Inport
  Add : Sum  Inputs=+-++
  Constant : Constant  Value=218.05
  Constant1 : Constant  Value=30129
  Constant2 : Constant  Value=3
  Constant3 : Constant  Value=61000
  Display : Display
  Gain : Gain  Gain=0.0066
  Gain1 : Gain  Gain=1.5533
  Math Function : Math  Operator=pow  SignedPower=on
  Math Function1 : Math  Operator=square  SignedPower=on
  Product : Product
  Saturation3 : Saturate  UpperLimit=60000  LowerLimit=30000
  Saturation6 : Saturate  UpperLimit=167  LowerLimit=60
  Scope : Scope
  PWCOUNT : Outport  VectorParamsAs1DForOutWhenUnconnected=off
  wires:
  Add/1 -> Saturation3/1
  U1/1 -> Saturation6/1
  Constant/1 -> Product/2
  Gain/1 -> Add/1
  Math Function/1 -> Gain/1
  Constant2/1 -> Math Function/2
  Math Function1/1 -> Gain1/1
  Gain1/1 -> Add/2
  Product/1 -> Add/3
  Constant1/1 -> Add/4
  Saturation6/1 -> Math Function/1, Math Function1/1, Product/1
  Saturation3/1 -> Display/1, Scope/1, PWCOUNT/1

== system REAL_THREE_TANK/Three tank sys/THREE_TANKS REALTIME_ PLANT/PUMPS AND VALVES/PUMP-40k-min ==
  note: p1 = 0.0047 p2 = -0.4981 p3 = 45.375 p4 = 37953
  U1 : Inport
  Add : Sum  Inputs=+-++
  Constant : Constant  Value=45.375
  Constant1 : Constant  Value=37953
  Constant2 : Constant  Value=3
  Constant3 : Constant  Value=61000
  Display : Display
  Gain : Gain  Gain=0.0047
  Gain1 : Gain  Gain=0.4981
  Math Function : Math  Operator=pow  SignedPower=on
  Math Function1 : Math  Operator=square  SignedPower=on
  Product : Product
  Saturation3 : Saturate  UpperLimit=60000  LowerLimit=30000
  Saturation6 : Saturate  UpperLimit=167  LowerLimit=60
  Scope : Scope
  PWCOUNT : Outport  VectorParamsAs1DForOutWhenUnconnected=off
  wires:
  Add/1 -> Saturation3/1
  U1/1 -> Saturation6/1
  Constant/1 -> Product/2
  Gain/1 -> Add/1
  Math Function/1 -> Gain/1
  Constant2/1 -> Math Function/2
  Math Function1/1 -> Gain1/1
  Gain1/1 -> Add/2
  Product/1 -> Add/3
  Constant1/1 -> Add/4
  Saturation6/1 -> Math Function/1, Math Function1/1, Product/1
  Saturation3/1 -> Display/1, Scope/1, PWCOUNT/1

== system REAL_THREE_TANK/Three tank sys/THREE_TANKS REALTIME_ PLANT/PUMPS AND VALVES/PUMP-final 3rd-order ==
  U1 : Inport
  Add : Sum  Inputs=+-++
  Constant : Constant  Value=595.22
  Constant1 : Constant  Value=1757.5
  Constant2 : Constant  Value=3
  Constant3 : Constant  Value=61000
  Display : Display
  Gain : Gain  Gain=0.0071
  Gain1 : Gain  Gain=2.9405
  Math Function : Math  Operator=pow  SignedPower=on
  Math Function1 : Math  Operator=square  SignedPower=on
  Product : Product
  Saturation3 : Saturate  UpperLimit=60000  LowerLimit=30000
  Saturation6 : Saturate  UpperLimit=230  LowerLimit=0
  Scope : Scope
  PWCOUNT : Outport  VectorParamsAs1DForOutWhenUnconnected=off
  wires:
  Add/1 -> Saturation3/1
  U1/1 -> Saturation6/1
  Constant/1 -> Product/2
  Gain/1 -> Add/1
  Math Function/1 -> Gain/1
  Constant2/1 -> Math Function/2
  Math Function1/1 -> Gain1/1
  Gain1/1 -> Add/2
  Product/1 -> Add/3
  Constant1/1 -> Add/4
  Saturation6/1 -> Math Function/1, Math Function1/1, Product/1
  Saturation3/1 -> Display/1, Scope/1, PWCOUNT/1

== system REAL_THREE_TANK/Three tank sys/THREE_TANKS REALTIME_ PLANT/PUMPS AND VALVES/PUMP-final-2nd-order ==
  U1 : Inport
  Add : Sum  Inputs=-++
  Constant : Constant  Value=4165.1
  Constant2 : Constant  Value=2
  Display : Display
  Gain : Gain  Gain=0.48
  Gain1 : Gain  Gain=378.33
  Math Function : Math  Operator=pow  SignedPower=on
  Saturation3 : Saturate  UpperLimit=65535  LowerLimit=0
  Saturation6 : Saturate  UpperLimit=188.5  LowerLimit=0
  Scope : Scope
  PWCOUNT : Outport  VectorParamsAs1DForOutWhenUnconnected=off
  wires:
  Gain/1 -> Add/1
  U1/1 -> Saturation6/1, Gain1/1
  Math Function/1 -> Gain/1
  Constant2/1 -> Math Function/2
  Saturation6/1 -> Math Function/1
  Saturation3/1 -> Display/1, Scope/1, PWCOUNT/1
  Gain1/1 -> Add/2
  Constant/1 -> Add/3
  Add/1 -> Saturation3/1

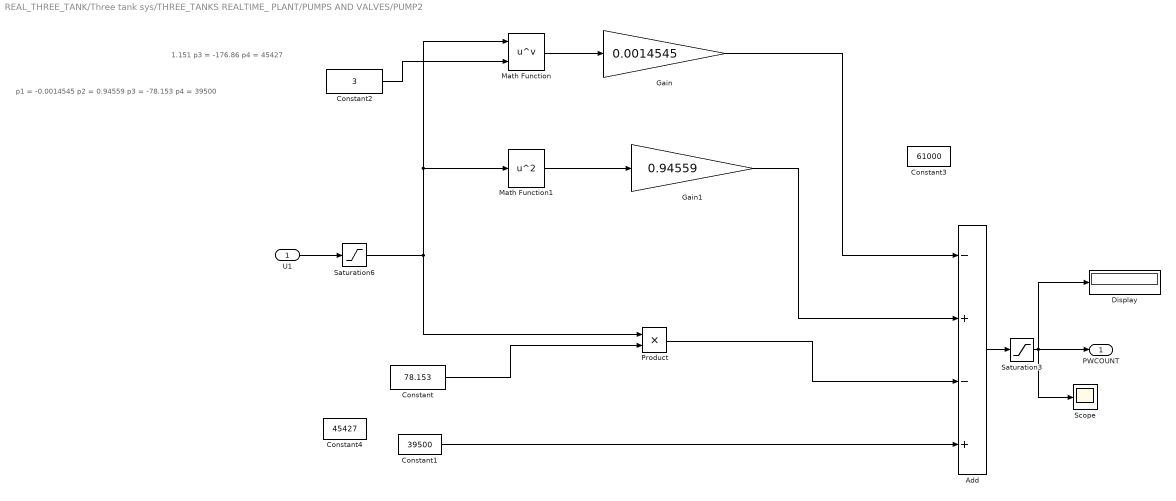
== system REAL_THREE_TANK/Three tank sys/THREE_TANKS REALTIME_ PLANT/PUMPS AND VALVES/PUMP2 ==
  note: 1.151 p3 = -176.86 p4 = 45427
  note: p1 = -0.0014545 p2 = 0.94559 p3 = -78.153 p4 = 39500
  U1 : Inport
  Add : Sum  Inputs=-+-+
  Constant : Constant  Value=78.153
  Constant1 : Constant  Value=39500
  Constant2 : Constant  Value=3
  Constant3 : Constant  Value=61000
  Constant4 : Constant  Value=45427
  Display : Display
  Gain : Gain  Gain=0.0014545
  Gain1 : Gain  Gain=0.94559
  Math Function : Math  Operator=pow  SignedPower=on
  Math Function1 : Math  Operator=square  SignedPower=on
  Product : Product
  Saturation3 : Saturate  UpperLimit=65535  LowerLimit=0
  Saturation6 : Saturate  UpperLimit=420  LowerLimit=0
  Scope : Scope
  PWCOUNT : Outport  VectorParamsAs1DForOutWhenUnconnected=off
  wires:
  Saturation3/1 -> PWCOUNT/1, Scope/1, Display/1
  Saturation6/1 -> Product/1, Math Function1/1, Math Function/1
  Constant1/1 -> Add/4
  Product/1 -> Add/3
  Gain1/1 -> Add/2
  Math Function1/1 -> Gain1/1
  Constant2/1 -> Math Function/2
  Math Function/1 -> Gain/1
  Gain/1 -> Add/1
  Constant/1 -> Product/2
  U1/1 -> Saturation6/1
  Add/1 -> Saturation3/1

== system REAL_THREE_TANK/Three tank sys/THREE_TANKS REALTIME_ PLANT/SENSORS/HEIGTH SENSOR1 ==
  pwC : Inport
  Add : Sum  Inputs=+-+
  Constant : Constant  Value=0.0752
  Constant1 : Constant  Value=246.42
  Constant2 : Constant  Value=0.06
  Display : Display
  Product : Product
  Scope : Scope
      settings: DataLoggingVariableName=ScopeData2
  H 1 : Outport  VectorParamsAs1DForOutWhenUnconnected=off
  wires:
  pwC/1 -> Product/1
  Constant/1 -> Product/2
  Product/1 -> Add/1
  Constant1/1 -> Add/2
  Add/1 -> Display/1, H 1/1, Scope/1
  Constant2/1 -> Add/3

== system REAL_THREE_TANK/Three tank sys/THREE_TANKS REALTIME_ PLANT/SENSORS/HEIGTH SENSOR2 ==
  PWC : Inport
  Constant : Constant  Value=0.0755
  Constant1 : Constant  Value=249.45
  Constant2 : Constant  Value=0.04
  Display : Display
  Product : Product
  Scope : Scope
  Subtract : Sum  Inputs=+-+
  H2 : Outport  VectorParamsAs1DForOutWhenUnconnected=off
  wires:
  Constant/1 -> Product/2
  PWC/1 -> Product/1
  Product/1 -> Subtract/1
  Constant1/1 -> Subtract/2
  Subtract/1 -> Scope/1, Display/1, H2/1
  Constant2/1 -> Subtract/3

== system REAL_THREE_TANK/Three tank sys/THREE_TANKS REALTIME_ PLANT/SENSORS/HEIGTH SENSOR3 ==
  PWC : Inport
  Constant : Constant  Value=0.0748
  Constant1 : Constant  Value=246.01
  Constant2 : Constant  Value=0
  Display : Display
  Product : Product
  Scope : Scope
  Subtract : Sum  Inputs=+-+
  H3 : Outport  VectorParamsAs1DForOutWhenUnconnected=off
  wires:
  PWC/1 -> Product/1
  Constant/1 -> Product/2
  Product/1 -> Subtract/1
  Constant1/1 -> Subtract/2
  Subtract/1 -> Display/1, Scope/1, H3/1
  Constant2/1 -> Subtract/3

== system REAL_THREE_TANK/Three tank sys/THREE_TANKS REALTIME_ PLANT/3 TANK  SYSTEM /RECEIVE/Subsystem1 ==
  In2 : Inport
  In3 : Inport  Port=2
  In4 : Inport  Port=3
  In5 : Inport  Port=4
  Constant : Constant  Value=48
  Constant1 : Constant  Value=0
  Gain1 : Gain  Gain=1000
  Gain2 : Gain  Gain=100
  Gain3 : Gain  Gain=10
  Gain4 : Gain
  Subtract{1..4} (4 alike) : Sum  Inputs=+-
  Subtract5 : Sum  Inputs=+++++
  Out1 : Outport  VectorParamsAs1DForOutWhenUnconnected=off
  wires:
  Constant1/1 -> Subtract5/1
  Constant/1 -> Subtract4/2, Subtract3/2, Subtract2/2, Subtract1/2
  Gain2/1 -> Subtract5/3
  Subtract1/1 -> Gain1/1
  Gain3/1 -> Subtract5/4
  Subtract4/1 -> Gain4/1
  Gain4/1 -> Subtract5/5
  In5/1 -> Subtract4/1
  In4/1 -> Subtract3/1
  Subtract3/1 -> Gain3/1
  Gain1/1 -> Subtract5/2
  Subtract2/1 -> Gain2/1
  Subtract5/1 -> Out1/1
  In3/1 -> Subtract2/1
  In2/1 -> Subtract1/1

== system REAL_THREE_TANK/Three tank sys/THREE_TANKS REALTIME_ PLANT/3 TANK  SYSTEM /RECEIVE/Subsystem2 ==
  In2 : Inport
  In3 : Inport  Port=2
  In4 : Inport  Port=3
  In5 : Inport  Port=4
  Constant : Constant  Value=48
  Constant1 : Constant  Value=0
  Gain1 : Gain  Gain=1000
  Gain2 : Gain  Gain=100
  Gain3 : Gain  Gain=10
  Gain4 : Gain
  Subtract{1..4} (4 alike) : Sum  Inputs=+-
  Subtract5 : Sum  Inputs=+++++
  Out1 : Outport  VectorParamsAs1DForOutWhenUnconnected=off
  wires:
  In2/1 -> Subtract1/1
  In3/1 -> Subtract2/1
  Subtract5/1 -> Out1/1
  Subtract2/1 -> Gain2/1
  Gain1/1 -> Subtract5/2
  Subtract3/1 -> Gain3/1
  In4/1 -> Subtract3/1
  In5/1 -> Subtract4/1
  Gain4/1 -> Subtract5/5
  Subtract4/1 -> Gain4/1
  Gain3/1 -> Subtract5/4
  Subtract1/1 -> Gain1/1
  Gain2/1 -> Subtract5/3
  Constant/1 -> Subtract1/2, Subtract2/2, Subtract3/2, Subtract4/2
  Constant1/1 -> Subtract5/1

== system REAL_THREE_TANK/Three tank sys/THREE_TANKS REALTIME_ PLANT/3 TANK  SYSTEM /RECEIVE/Subsystem4 ==
  In2 : Inport
  In3 : Inport  Port=2
  In4 : Inport  Port=3
  In5 : Inport  Port=4
  Constant : Constant  Value=48
  Constant1 : Constant  Value=0
  Gain1 : Gain  Gain=1000
  Gain2 : Gain  Gain=100
  Gain3 : Gain  Gain=10
  Gain4 : Gain
  Subtract{1..4} (4 alike) : Sum  Inputs=+-
  Subtract5 : Sum  Inputs=+++++
  Out1 : Outport  VectorParamsAs1DForOutWhenUnconnected=off
  wires:
  Constant1/1 -> Subtract5/1
  Constant/1 -> Subtract4/2, Subtract3/2, Subtract2/2, Subtract1/2
  Gain2/1 -> Subtract5/3
  Subtract1/1 -> Gain1/1
  Gain3/1 -> Subtract5/4
  Subtract4/1 -> Gain4/1
  Gain4/1 -> Subtract5/5
  In5/1 -> Subtract4/1
  In4/1 -> Subtract3/1
  Subtract3/1 -> Gain3/1
  Gain1/1 -> Subtract5/2
  Subtract2/1 -> Gain2/1
  Subtract5/1 -> Out1/1
  In3/1 -> Subtract2/1
  In2/1 -> Subtract1/1

== matlab function REAL_THREE_TANK/Three tank sys/THREE_TANKS REALTIME_ PLANT/3 TANK  SYSTEM /SEND/MATLAB Function1 ==
  data: real_ht input; y output; set_ht input; set_min input; pwm_in input
function y = fcn(real_ht,set_ht,set_min,pwm_in)
      temp = pwm_in;
if (real_ht >= set_ht)
      temp = set_min;
 end
       
y = temp;

== matlab function REAL_THREE_TANK/Three tank sys/THREE_TANKS REALTIME_ PLANT/3 TANK  SYSTEM /SEND/MATLAB Function3 ==
  data: real_ht input; y output; set_ht input; set_min input; Valvm_in input
function y = fcn(real_ht,set_ht,set_min,Valvm_in)
      temp = Valvm_in;
if (real_ht >= set_ht)
      temp = set_min;
 end
       
y = temp;

== matlab function REAL_THREE_TANK/Three tank sys/THREE_TANKS REALTIME_ PLANT/3 TANK  SYSTEM /SEND/MATLAB Function4 ==
  data: real_ht input; y output; set_ht input; set_min input; Valvm_in input
function y = fcn(real_ht,set_ht,set_min,Valvm_in)
      temp = Valvm_in;
if (real_ht >= set_ht)
      temp = set_min;
 end
       
y = temp;

== matlab function REAL_THREE_TANK/Three tank sys/THREE_TANKS REALTIME_ PLANT/3 TANK  SYSTEM /SEND/MATLAB Function5 ==
  data: real_ht input; y output; set_ht input; set_min input; Valvm_in input
function y = fcn(real_ht,set_ht,set_min,Valvm_in)
      temp = Valvm_in;
if (real_ht >= set_ht)
      temp = set_min;
 end
       
y = temp;

== matlab function REAL_THREE_TANK/NMPC/NMPC  ==
  data: uopt output; y_pred output; fcost output size=[1,1]; Ecount output; exitflag output; xPx output; Tconst output; y_set input; ypast input; yo input; tp input; ts input; dist input; upast input; uo input; u_set input; ho input; hk output; modelName input
function [uopt, y_pred, fcost, Ecount, exitflag, xPx, Tconst, hk] = nmpc(y_set, ypast, yo, tp, ts, dist, upast, uo, u_set, ho, modelName)
uopt = [0;0;0];
fcost = 0;
y_pred = [0;0;0];
u_reg = [upast(1) upast(2), upast(3);uo(1) uo(2),uo(3)];
y_reg =[ypast';yo'];
Ecount = 0 ;
exitflag = Inf ;
xPx = 0 ;
Tconst = 0 ;
hk = ho;
h1ss=y_set(1) ; h2ss=y_set(2) ; h3ss=y_set(3) ;
u1ss=u_set(1) ; u2ss=u_set(2) ; u3ss = u_set(3);
rhox = 20;
rhou=10;
Wy = [1/h1ss, 1/h2ss, 1/h3ss]*rhox;
% FIX 1: no penalty on (u - u_set)
Wu    = [0, 0, 0];
Wdu   = [1/u1ss,10/u2ss, 10/u3ss]*rhou;
Wuerr = [0, 0, 0];
P1 =[
    0.3408    0.1556    0.0754;
    0.1556    0.4888    0.2504;
    0.0754    0.2504    0.6810;];
alpha1 = 20.4206;
P=P1;
alpha = alpha1*rhox;
nu = tp(1);
ny = tp(2);
Nu = tp(3);
Np = tp(4);
bounds = struct();
bounds.ymin =[0.1 ,0.1, 0.1];
bounds.ymax =[35 35 35];
% FIX 2: input bounds = PINN training range
bounds.u_min = [55,  0.17, 0.11];
bounds.u_max = [148, 1.00, 0.87];
du = [10, 0.1, 0.1];
bounds.du_min =  -du;
bounds.du_max = du;
params = struct();
params.y_set = y_set;
params.u_set = u_set;
params.nu = nu;
params.ny = ny;
params.Nu = Nu;
params.Np = Np;
params.Wy = Wy;
params.Wdu = Wdu;
params.Wu = Wu;
params.Wuerr =Wuerr;
params.ts = ts;
params.P = P;
params.alpha = alpha;
params.modelName = modelName;
params.bounds = bounds;
params.dist = dist;
coder.extrinsic('get_control_input');
[uopt, y_pred, hk, fval, exitflag, elapsed, ~, ~] = get_control_input(y_reg, u_reg, ho, params);
% FIX 3: show the raw PINN prediction on the scope
y_pred = y_pred(:) - dist(:);
fcost = fval;
Ecount = elapsed ;
end

== matlab function REAL_THREE_TANK/safety_guard ==
  data: u input; u_safe output; h input
function u_safe = safety_guard(u, h)
%#codegen
% Hardware guard: stops the pump and opens both valves if any tank is
% near overflow. Latches until every level drops below H_RESET.
H_TRIP  = 33;    % cm - trip level (tanks are 35 cm)
H_RESET = 30;    % cm - release level
U_MIN = [55;  0.17; 0.11];
U_MAX = [148; 1.00; 0.87];

persistent tripped
if isempty(tripped)
    tripped = false;
end

if any(h(:) > H_TRIP)
    tripped = true;
elseif all(h(:) < H_RESET)
    tripped = false;
end

if tripped
    u_safe = [0; 1; 1];          % pump off, both valves fully open
else
    u_safe = min(max(u(:), U_MIN), U_MAX);
end
end

== matlab function REAL_THREE_TANK/Three tank sys/THREE_TANKS REALTIME_ PLANT/3 TANK  SYSTEM /MATLAB Function ==
  data: u input; y output
function y = fcn(u)
 persistent pp;
 if isempty(pp)
     %system just starting
   pp = 0;
   temp = 0;
 end
 temp = 0;
 if (u == 0)&&(pp == 1)  %detect falling edge
    temp = 1; 
 end
 pp = u;  %store last value
y = temp;
